simulink model "AC_DC_CONVERTOR"  (R2024b)
settings: Solver=VariableStepAuto  StartTime=0.0  StopTime=10.0  RelTol=1e-3
libraries: fl_lib x10, nesl_utility x5, spsThyristorLib x4, spsVoltageMeasurementLib x3, simulink x3, spsSeriesRLCBranchLib x2, spsCurrentMeasurementLib x1, spsControlledVoltageSourceLib x1, ee_lib x1, sps_lib x1
settings Model: VariantFading=off  Creator=Abdal  LastModifiedBy=Abdal
settings DebuggingCC: AlgebraicLoopMsg=none

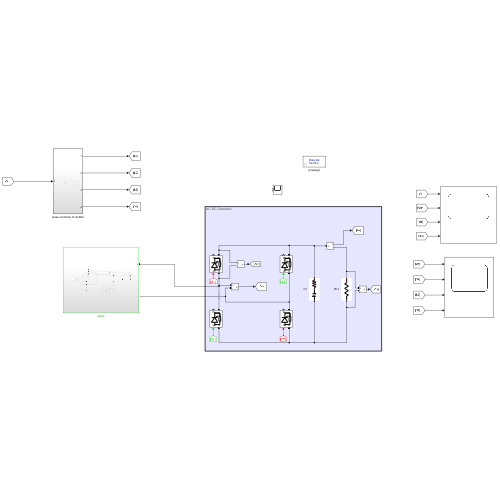
[thumbnail: Simulink's stored preview of the top-level diagram]
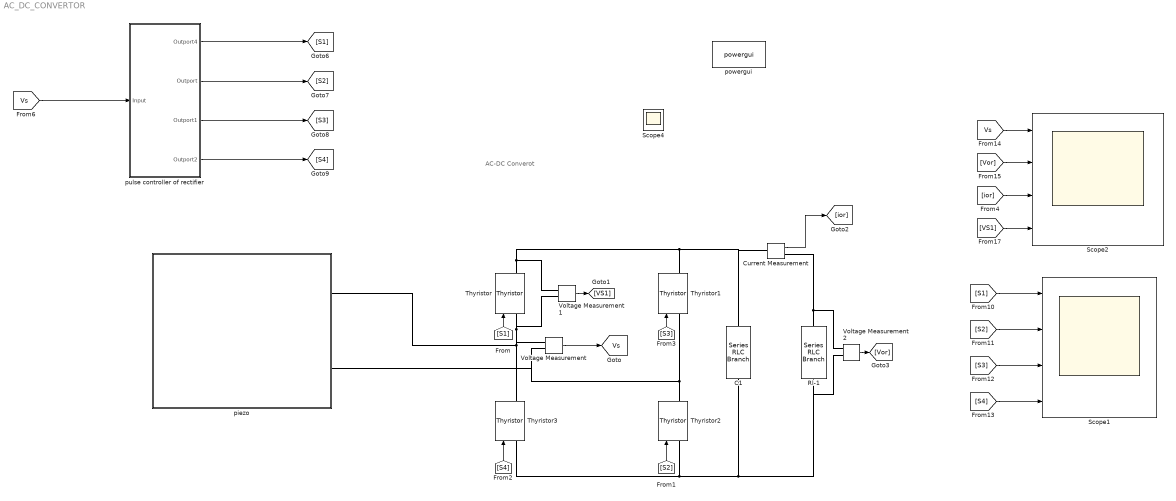
== system AC_DC_CONVERTOR ==
  note: AC-DC Converot
  C1 : spsSeriesRLCBranchLib/Series RLC Branch  LConnTagsString=__new0  RConnTagsString=__new0  BranchType=RC  Resistance=1  Inductance=1e-3  SetiL0=off  InitialCurrent=0  Capacitance=4500  Setx0=off  InitialVoltage=0  Measurements=None
  Current Measurement : spsCurrentMeasurementLib/Current Measurement  PhasorSimulation=off  OutputType=Complex  PSBequivalent=0
  Rl-1 : spsSeriesRLCBranchLib/Series RLC Branch  LConnTagsString=__new0  RConnTagsString=__new0  BranchType=R  Resistance=200  Inductance=1e-3  SetiL0=off  InitialCurrent=0  Capacitance=1e-6  Setx0=off  InitialVoltage=0  Measurements=None
  Scope1 : Scope  NumInputPorts=4
  Scope2 : Scope  NumInputPorts=4
  Scope4 : Scope
  Thyristor : spsThyristorLib/Thyristor  Ron=100  Lon=0  Vf=24  IC=0  Rs=100  Cs=4500  Measurements=on
  Thyristor1 : spsThyristorLib/Thyristor  Ron=0.001  Lon=0  Vf=24  IC=0  Rs=100  Cs=4500  Measurements=on
  Thyristor2 : spsThyristorLib/Thyristor  Ron=0.001  Lon=0  Vf=24  IC=0  Rs=100  Cs=4500  Measurements=on
  Thyristor3 : spsThyristorLib/Thyristor  Ron=0.001  Lon=0  Vf=24  IC=0  Rs=100  Cs=4500  Measurements=on
  Voltage Measurement : spsVoltageMeasurementLib/Voltage Measurement  PhasorSimulation=off  OutputType=Complex  PSBequivalent=0
  Voltage Measurement1 : spsVoltageMeasurementLib/Voltage Measurement  PhasorSimulation=off  OutputType=Complex  PSBequivalent=0
  Voltage Measurement2 : spsVoltageMeasurementLib/Voltage Measurement  PhasorSimulation=off  OutputType=Complex  PSBequivalent=0
  piezo : Subsystem
  powergui : sps_lib/powergui  Priority=1  SimulationMode=Discrete  SampleTime=50e-6  frequency=60  Iterations=50  frequencyindice=0  Pbase=100e6  ErrMax=1e-4  UnitsV=kV  UnitsW=MW  buscounter=0  FunctionMessages=off  echomessages=off  EnableUseOfTLC=off  CurrentSourceSwitches=off  DisableSnubberDevices=off  DisableRonSwitches=off  DisableVfSwitches=off  DisplayEquations=off  AutomaticDiscreteSolvers=off  SolverType=Tustin/Backward Euler (TBE)  Interpol=off  ExternalGateDelay=off  methode=off  Ts=100  x0status=blocks  SPID=on  SwTol=0  HookPort=off  NonlinearTolerance=1e-4  nMaxIteration=100  ContinueOnMaxIteration=off  RestoreLinks=warning  ResistiveCurrentMeasurement=off  Frange=[0:2:500]  Ylog=off  Xlog=on  ShowGrid=off  save=off  variable=ZData  structure=0  ZoomFFT=off  StartTime=0.0  cycles=1  DisplayStyle=1  fundamental=60  FreqAxis=off  MaxFrequency=1000  frequencyindicesteady=1  RmsSteady=1  display=off
  pulse controller of rectifier : Subsystem
  tag scope: Vs=global
  wires:
  Voltage Measurement/1 -> [Vs]
  [S1] -> Thyristor/1
  [S2] -> Thyristor2/1
  [S3] -> Thyristor1/1
  [S4] -> Thyristor3/1
  Voltage Measurement1/1 -> [VS1]
  Voltage Measurement2/1 -> [Vor]
  [Vs] -> pulse controller of rectifier/1(Input)
  pulse controller of rectifier/4(Outport2) -> [S4]
  [S1] -> Scope1/1
  [S2] -> Scope1/2
  [S3] -> Scope1/3
  [S4] -> Scope1/4
  pulse controller of rectifier/1(Outport4) -> [S1]
  pulse controller of rectifier/2(Outport) -> [S2]
  pulse controller of rectifier/3(Outport1) -> [S3]
  [Vs] -> Scope2/1
  [Vor] -> Scope2/2
  [ior] -> Scope2/3
  [VS1] -> Scope2/4
  Current Measurement/1 -> [ior]
  connections:
  Thyristor3/RConn1 -- Voltage Measurement/LConn1 -- Voltage Measurement1/LConn2 -- Thyristor/LConn1 -- piezo/LConn1
  Thyristor/RConn1 -- Voltage Measurement1/LConn1 -- Current Measurement/LConn1 -- C1/LConn1 -- Thyristor1/RConn1
  Thyristor1/LConn1 -- piezo/LConn2 -- Voltage Measurement/LConn2 -- Thyristor2/RConn1
  Thyristor3/LConn1 -- Thyristor2/LConn1 -- Voltage Measurement2/LConn2 -- Rl-1/RConn1 -- C1/RConn1
  Rl-1/LConn1 -- Current Measurement/RConn1 -- Voltage Measurement2/LConn1

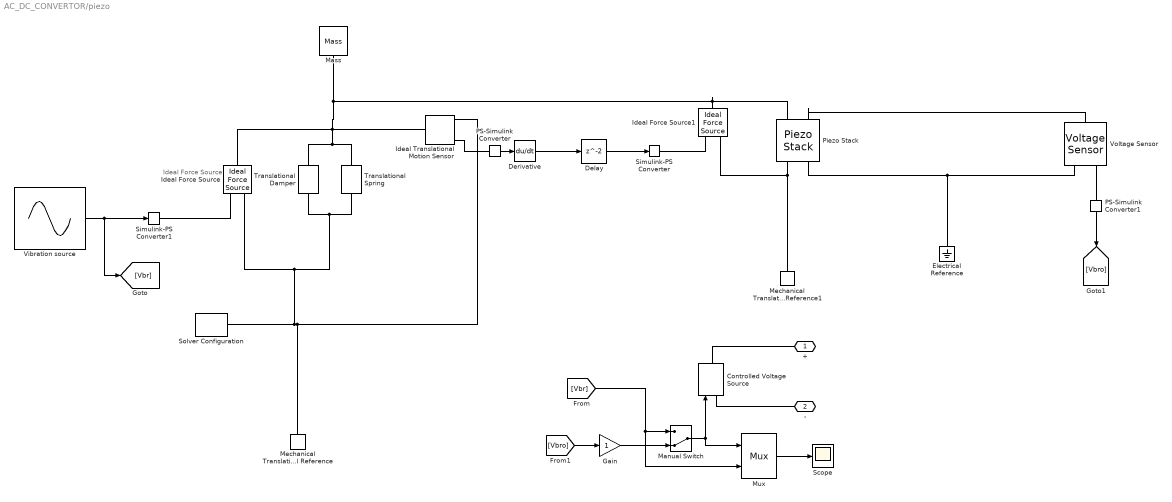
== system AC_DC_CONVERTOR/piezo ==
  note: Ideal Force Source
  Controlled Voltage Source : spsControlledVoltageSourceLib/Controlled Voltage Source  Initialize=on  Source_Type=AC  Amplitude=200  Phase=0  Frequency=4500  Measurements=None
  Delay : Delay
  Derivative : Derivative
  Electrical Reference : fl_lib/Electrical/Electrical Elements/Electrical Reference
  Gain : Gain
  Ideal Force Source : fl_lib/Mechanical/Mechanical Sources/Ideal Force Source
  Ideal Force Source1 : fl_lib/Mechanical/Mechanical Sources/Ideal Force Source
  Ideal Translational Motion Sensor : fl_lib/Mechanical/Mechanical Sensors/Ideal Translational Motion Sensor  reference=foundation.enum.MeasurementReference.difference  acceleration_port=false  velocity_port=true  position_port=true  offset=0 m
  Manual Switch : ManualSwitch  CurrentSetting=0
  Mass : fl_lib/Mechanical/Translational Elements/Mass  mass=3.6 kg  num_ports=foundation.enum.numPorts2.one  v_specify=off  v_priority=High  v=0 m/s  v_nominal_specify=off  v_nominal_value=1  v_nominal_unit=m/s  f_specify=off  f_priority=None  f=0 N  f_nominal_specify=off  f_nominal_value=1  f_nominal_unit=N
  Mechanical Translational Reference : fl_lib/Mechanical/Translational Elements/Mechanical Translational Reference
  Mechanical Translational Reference1 : fl_lib/Mechanical/Translational Elements/Mechanical Translational Reference
  Mux : Mux  Inputs=2
      settings: DisplayOption=signals
  PS-Simulink Converter : nesl_utility/PS-Simulink Converter  PhysicalDomain=network_engine_domain  SubClassName=ps_output  LeftPortType=input  RightPortType=output  PseudoPeriodic=off  Frequencies=[]  VectorFormat=inherit  Unit=inherit  AffineConversion=off
  PS-Simulink Converter1 : nesl_utility/PS-Simulink Converter  PhysicalDomain=network_engine_domain  SubClassName=ps_output  LeftPortType=input  RightPortType=output  PseudoPeriodic=off  Frequencies=[]  VectorFormat=inherit  Unit=inherit  AffineConversion=off
  Piezo Stack : ee_lib/Electromechanical/Mechatronic Actuators/Piezo Stack  param=ee.enum.actuators.datasheetOrMaterialProps.datasheet  A=100 mm^2  L0=36 mm  dt=0.3 mm  NL=50  dL0=0.038 mm  F0=3800 N  V0=120 V  C0=13 uF  d=500e-12 m/V  epsilon=2.1240e-08 F/m  s=19e-12 m^2/N  paramDyn=ee.enum.actuators.datasheetOrMaterialProps.datasheet  f=inf kHz  Qm=inf  Mass=0 g  lam=0 N*s/m  force_specify=off  force_priority=None  force=0 N  force_nominal_specify=off  force_nominal_value=1  force_nominal_unit=N  vel_specify=off  vel_priority=None  vel=0 mm/s  vel_nominal_specify=off  vel_nominal_value=1  vel_nominal_unit=mm/s  x_specify=off  x_priority=None  x=0 mm  x_nominal_specify=off  x_nominal_value=1  x_nominal_unit=mm  v_specify=off  v_priority=None  v=0 V  v_nominal_specify=off  v_nominal_value=1  v_nominal_unit=V
      settings: InternalSimscapePortConfiguration="{\"Bottom\":[],\"Left\":[{\"id\":\"p\",\"label\":\"+\",\"type\":\"foundation.electrical.electrical\"},{\"id\":\"R\",\"label\":\"R\",\"type\":\"foundation.mechanical.translational.translational\"}],\"Right\":[{\"id\":\"n\",\"label\":\"-\",\"type\":\"foundation.electrical.electrical\"},{\"id\":\"C\",\"label\":\"C\",\"type\":\"foundation.mechanical.translational.translational\"}],\"Top\":[]}"
  Scope : Scope
  Simulink-PS Converter : nesl_utility/Simulink-PS Converter  PhysicalDomain=network_engine_domain  SubClassName=ps_input  LeftPortType=input  RightPortType=output  PseudoPeriodic=off  Frequencies=[]  NoiseDistribution=none  NoiseParameters=[]  Unit=1  AffineConversion=off  FilteringAndDerivatives=provide  SimscapeFilterOrder=1  InputFilterTimeConstant=0.001  UdotUserProvided=0
  Simulink-PS Converter1 : nesl_utility/Simulink-PS Converter  PhysicalDomain=network_engine_domain  SubClassName=ps_input  LeftPortType=input  RightPortType=output  PseudoPeriodic=off  Frequencies=[]  NoiseDistribution=none  NoiseParameters=[]  Unit=1  AffineConversion=off  FilteringAndDerivatives=provide  SimscapeFilterOrder=1  InputFilterTimeConstant=0.001  UdotUserProvided=0
  Solver Configuration : nesl_utility/Solver Configuration  PhysicalDomain=network_engine_domain  SubClassName=solver  LeftPortType=input  RightPortType=generic  Tones=[]  Harmonics=[]  SimulateNoise=off  Profile=off  UseLocalSampling=off  EnableSwitchedLinearOptims=on  FrequencyDomain=off  UseCCode=off  RelTol=0.001  AbsTol=0.001  MinStep=1e-09  ToWorkspace=off  RevertToSquareIcSolve=off  NumHomotopyIterations=100  PhasorMode=off  PhasorModeNumHarmonics=1  ConsistencySolver=NEWTON_XTOL_AFTER_FTOL  IndexReductionMethod=DerivativeReplacement  DoDC=off  ResidualTolerance=1e-09  ConsistencyTolSource=GLOBAL  ConsistencyAbsTol=0.001  ConsistencyRelTol=0.001  ConsistencyTolFactor=0.001  UseLocalSolver=off  LocalSolverChoice=NE_BACKWARD_EULER_ADVANCER  ResolveIndetEquations=on  FunctionEvalNumThread=1  LocalSolverSampleTime=0.001  DoFixedCost=off  MaxNonlinIter=3  MaxModeIter=2  ComputeImpulses=off  ImpulseIterations=2  LinearAlgebra=auto  LinearAlgebraNumThread=0  EquationFormulation=NE_TIME_EF  DelaysMemoryBudget=1024  AutomaticFiltering=on  FilteringTimeConstant=0.001  PartitionStorageMethod=AS_NEEDED  PartitionMemoryBudget=1024  PartitionMethod=ROBUST  MultibodyUseLocalSolver=off  MultibodyLocalSolverChoice=ODE1  MultibodyLocalSolverSampleTime=0.001
  Translational Damper : fl_lib/Mechanical/Translational Elements/Translational Damper  D=100 N*s/m  v_specify=off  v_priority=None  v=0 m/s  v_nominal_specify=off  v_nominal_value=1  v_nominal_unit=m/s  f_specify=off  f_priority=None  f=0 N  f_nominal_specify=off  f_nominal_value=1  f_nominal_unit=N
  Translational Spring : fl_lib/Mechanical/Translational Elements/Translational Spring  spr_rate=400 N/m  v_specify=off  v_priority=None  v=0 m/s  v_nominal_specify=off  v_nominal_value=1  v_nominal_unit=m/s  f_specify=off  f_priority=None  f=0 N  f_nominal_specify=off  f_nominal_value=1  f_nominal_unit=N  x_specify=off  x_priority=High  x=0 m  x_nominal_specify=off  x_nominal_value=1  x_nominal_unit=m
  Vibration source : Sin  Amplitude=200  Frequency=50  SampleTime=0
  Voltage Sensor : fl_lib/Electrical/Electrical Sensors/Voltage Sensor
  + : PMIOPort  Side=Left
  - : PMIOPort  Port=2  Side=Left
  wires:
  PS-Simulink Converter/1 -> Derivative/1
  Derivative/1 -> Delay/1
  Vibration source/1 -> [Vbr], Simulink-PS Converter1/1
  PS-Simulink Converter1/1 -> [Vbro]
  [Vbro] -> Gain/1
  Manual Switch/1 -> Mux/1, Controlled Voltage Source/1
  [Vbr] -> Mux/2, Manual Switch/1
  Gain/1 -> Manual Switch/2
  Mux/1 -> Scope/1
  Delay/1 -> Simulink-PS Converter/1
  connections:
  Translational Damper/LConn1 -- Piezo Stack/LConn2 -- Ideal Force Source1/LConn1 -- Mass/LConn1 -- Ideal Force Source/LConn1 -- Ideal Translational Motion Sensor/LConn1 -- Translational Spring/LConn1
  Translational Damper/RConn1 -- Ideal Translational Motion Sensor/RConn1 -- Mechanical Translational Reference/LConn1 -- Solver Configuration/RConn1 -- Ideal Force Source/RConn2 -- Translational Spring/RConn1
  Mechanical Translational Reference1/LConn1 -- Ideal Force Source1/RConn2 -- Piezo Stack/RConn2
  Piezo Stack/LConn1 -- Voltage Sensor/LConn1
  Piezo Stack/RConn1 -- Electrical Reference/LConn1 -- Voltage Sensor/RConn2
  PS-Simulink Converter/LConn1 -- Ideal Translational Motion Sensor/RConn3
  Simulink-PS Converter/RConn1 -- Ideal Force Source1/RConn1
  Simulink-PS Converter1/RConn1 -- Ideal Force Source/RConn1
  PS-Simulink Converter1/LConn1 -- Voltage Sensor/RConn1
  Controlled Voltage Source/RConn1 -- +/RConn1
  Controlled Voltage Source/LConn1 -- -/RConn1

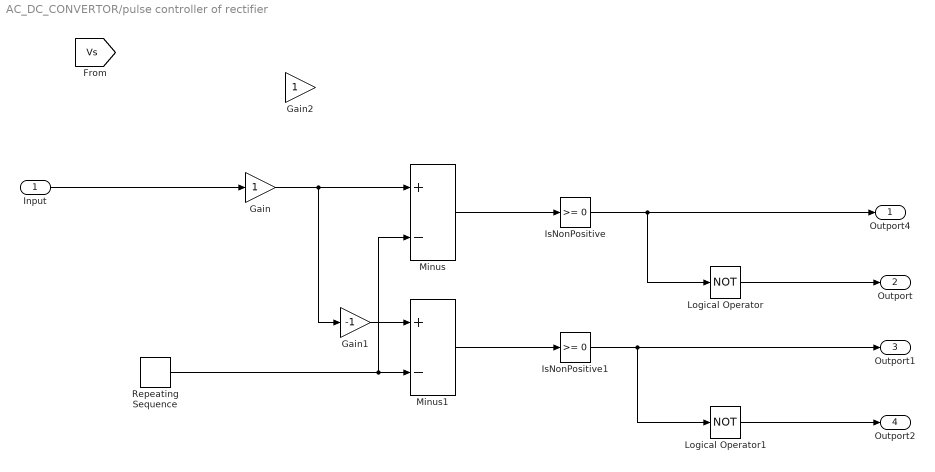
== system AC_DC_CONVERTOR/pulse controller of rectifier ==
  Input : Inport
  Gain : Gain
  Gain1 : Gain  Gain=-1
  Gain2 : Gain
  IsNonPositive : simulink/Logic and Bit Operations/Compare To Zero  relop=>=  OutDataTypeStr=boolean
      settings: LibrarySourceBlock=|
      | simulink/Quick Insert/Logic and Bit
      | Operations/IsNonPositive
  IsNonPositive1 : simulink/Logic and Bit Operations/Compare To Zero  relop=>=  OutDataTypeStr=boolean
      settings: LibrarySourceBlock=|
      | simulink/Quick Insert/Logic and Bit
      | Operations/IsNonPositive
  Logical Operator : Logic  Operator=NOT  AllPortsSameDT=off  OutDataTypeStr=boolean
  Logical Operator1 : Logic  Operator=NOT  AllPortsSameDT=off  OutDataTypeStr=boolean
  Minus : Sum  Inputs=+-
  Minus1 : Sum  Inputs=+-
  Repeating Sequence : simulink/Sources/Repeating Sequence  rep_seq_t=[0 2]  rep_seq_y=[0 2]
  Outport4 : Outport
  Outport : Outport  Port=2
  Outport1 : Outport  Port=3
  Outport2 : Outport  Port=4
  wires:
  Gain/1 -> Gain1/1, Minus/1
  Gain1/1 -> Minus1/1
  Repeating Sequence/1 -> Minus/2, Minus1/2
  Minus/1 -> IsNonPositive/1
  Minus1/1 -> IsNonPositive1/1
  IsNonPositive/1 -> Outport4/1, Logical Operator/1
  IsNonPositive1/1 -> Outport1/1, Logical Operator1/1
  Logical Operator/1 -> Outport/1
  Logical Operator1/1 -> Outport2/1
  Input/1 -> Gain/1
